simulink model "FW_SkySurfer_HIL"  (R2026b)
settings: Solver=ode4  StopTime=inf  FixedStep=Thil  EnableMultiTasking=on
PreLoadFcn:
  | % Load this folder's HIL settings and MAVLink Bus types (not another project's).
  | run(fullfile(fileparts(get_param(bdroot,'FileName')),'PX4_HIL_preload.m'));
InitFcn:
  | % Record the model first: loading libraries can change the current diagram.
  | assignin('base','lastRunModel',bdroot);
  | % Rebuild HIL settings/Bus types (also after clear all), then aircraft data.
  | hilModelFolder = fileparts(get_param(lastRunModel,'FileName'));
  | run(fullfile(hilModelFolder,'PX4_HIL_preload.m'));
  | run(fullfile(hilModelFolder,'FW_SkySurfer_InitialFunction.m'));
  | clear hilModelFolder
values from neighbouring files (symbols this model uses):
  Aeroelasticity_AIL = [   5   15]    [FW_SkySurfer_InitialFunction.m]
  Aeroelasticity_ELE = [   5   15]    [FW_SkySurfer_InitialFunction.m]
  Aeroelasticity_Gain_AIL = [ 0.8  0.5]    [FW_SkySurfer_InitialFunction.m]
  Aeroelasticity_Gain_ELE = [ 0.9  0.6]    [FW_SkySurfer_InitialFunction.m]
  Aeroelasticity_Gain_RUD = [ 0.9  0.6]    [FW_SkySurfer_InitialFunction.m]
  Aeroelasticity_RUD = [   5   15]    [FW_SkySurfer_InitialFunction.m]
  alpha_avl = [-10 -5 0 5 10 15]    [import_aerostates_avl.m]
  AoA = [-10 -5 0 5 10 15]    [import_aerostates_vsp.m]
  AoS = [-10 0 10]    [import_aerostates_vsp.m]
  b = 1.41    [FW_SkySurfer_InitialFunction.m]
  beta_avl = [-10 -5 0 5 10]    [import_aerostates_avl.m]
  C_wgrp = struct()    [import_aerostates_vsp.m]
  cbar = 0.20    (= 0.2)    [FW_SkySurfer_InitialFunction.m]
  CD_fix_AVL = 0.075    [FW_SkySurfer_InitialFunction.m]
  CD_fix_VSP = 0.065    [FW_SkySurfer_InitialFunction.m]
  CDd01 = zeros(length(mach_avl), length(alpha_avl), length(beta_avl))    [import_aerostates_avl.m]
  CDd02 = zeros(length(mach_avl), length(alpha_avl), length(beta_avl))    [import_aerostates_avl.m]
  CDd03 = zeros(length(mach_avl), length(alpha_avl), length(beta_avl))    [import_aerostates_avl.m]
  CDd04 = zeros(length(mach_avl), length(alpha_avl), length(beta_avl))    [import_aerostates_avl.m]
  CDp = zeros(length(mach_avl), length(alpha_avl), length(beta_avl))    [import_aerostates_avl.m]
  CDq = zeros(length(mach_avl), length(alpha_avl), length(beta_avl))    [import_aerostates_avl.m]
  CDr = zeros(length(mach_avl), length(alpha_avl), length(beta_avl))    [import_aerostates_avl.m]
  CDtot = zeros(length(mach_avl), length(alpha_avl), length(beta_avl))    [import_aerostates_avl.m]
  CG_m = [0.330, 0, 0]    [FW_SkySurfer_InitialFunction.m]
  CLd01 = zeros(length(mach_avl), length(alpha_avl), length(beta_avl))    [import_aerostates_avl.m]
  Cld01 = zeros(length(mach_avl), length(alpha_avl), length(beta_avl))    [import_aerostates_avl.m]
  CLd02 = zeros(length(mach_avl), length(alpha_avl), length(beta_avl))    [import_aerostates_avl.m]
  Cld02 = zeros(length(mach_avl), length(alpha_avl), length(beta_avl))    [import_aerostates_avl.m]
  CLd03 = zeros(length(mach_avl), length(alpha_avl), length(beta_avl))    [import_aerostates_avl.m]
  Cld03 = zeros(length(mach_avl), length(alpha_avl), length(beta_avl))    [import_aerostates_avl.m]
  CLd04 = zeros(length(mach_avl), length(alpha_avl), length(beta_avl))    [import_aerostates_avl.m]
  Cld04 = zeros(length(mach_avl), length(alpha_avl), length(beta_avl))    [import_aerostates_avl.m]
  CLp = zeros(length(mach_avl), length(alpha_avl), length(beta_avl))    [import_aerostates_avl.m]
  Clp = zeros(length(mach_avl), length(alpha_avl), length(beta_avl))    [import_aerostates_avl.m]
  CLq = zeros(length(mach_avl), length(alpha_avl), length(beta_avl))    [import_aerostates_avl.m]
  Clq = zeros(length(mach_avl), length(alpha_avl), length(beta_avl))    [import_aerostates_avl.m]
  CLr = zeros(length(mach_avl), length(alpha_avl), length(beta_avl))    [import_aerostates_avl.m]
  Clr = zeros(length(mach_avl), length(alpha_avl), length(beta_avl))    [import_aerostates_avl.m]
  CLtot = zeros(length(mach_avl), length(alpha_avl), length(beta_avl))    [import_aerostates_avl.m]
  Cltot = zeros(length(mach_avl), length(alpha_avl), length(beta_avl))    [import_aerostates_avl.m]
  Cmd01 = zeros(length(mach_avl), length(alpha_avl), length(beta_avl))    [import_aerostates_avl.m]
  Cmd02 = zeros(length(mach_avl), length(alpha_avl), length(beta_avl))    [import_aerostates_avl.m]
  Cmd03 = zeros(length(mach_avl), length(alpha_avl), length(beta_avl))    [import_aerostates_avl.m]
  Cmd04 = zeros(length(mach_avl), length(alpha_avl), length(beta_avl))    [import_aerostates_avl.m]
  Cmp = zeros(length(mach_avl), length(alpha_avl), length(beta_avl))    [import_aerostates_avl.m]
  Cmq = zeros(length(mach_avl), length(alpha_avl), length(beta_avl))    [import_aerostates_avl.m]
  Cmr = zeros(length(mach_avl), length(alpha_avl), length(beta_avl))    [import_aerostates_avl.m]
  Cmtot = zeros(length(mach_avl), length(alpha_avl), length(beta_avl))    [import_aerostates_avl.m]
  Cnd01 = zeros(length(mach_avl), length(alpha_avl), length(beta_avl))    [import_aerostates_avl.m]
  Cnd02 = zeros(length(mach_avl), length(alpha_avl), length(beta_avl))    [import_aerostates_avl.m]
  Cnd03 = zeros(length(mach_avl), length(alpha_avl), length(beta_avl))    [import_aerostates_avl.m]
  Cnd04 = zeros(length(mach_avl), length(alpha_avl), length(beta_avl))    [import_aerostates_avl.m]
  Cnp = zeros(length(mach_avl), length(alpha_avl), length(beta_avl))    [import_aerostates_avl.m]
  Cnq = zeros(length(mach_avl), length(alpha_avl), length(beta_avl))    [import_aerostates_avl.m]
  Cnr = zeros(length(mach_avl), length(alpha_avl), length(beta_avl))    [import_aerostates_avl.m]
  Cntot = zeros(length(mach_avl), length(alpha_avl), length(beta_avl))    [import_aerostates_avl.m]
  CYd01 = zeros(length(mach_avl), length(alpha_avl), length(beta_avl))    [import_aerostates_avl.m]
  CYd02 = zeros(length(mach_avl), length(alpha_avl), length(beta_avl))    [import_aerostates_avl.m]
  CYd03 = zeros(length(mach_avl), length(alpha_avl), length(beta_avl))    [import_aerostates_avl.m]
  CYd04 = zeros(length(mach_avl), length(alpha_avl), length(beta_avl))    [import_aerostates_avl.m]
  CYp = zeros(length(mach_avl), length(alpha_avl), length(beta_avl))    [import_aerostates_avl.m]
  CYq = zeros(length(mach_avl), length(alpha_avl), length(beta_avl))    [import_aerostates_avl.m]
  CYr = zeros(length(mach_avl), length(alpha_avl), length(beta_avl))    [import_aerostates_avl.m]
  CYtot = zeros(length(mach_avl), length(alpha_avl), length(beta_avl))    [import_aerostates_avl.m]
  del_z = 0    [FW_SkySurfer_InitialFunction.m]
  g = 9.80665    [FW_SkySurfer_InitialFunction.m]
  H0 = 1000 * convlength(1, 'ft', 'm')    [FW_SkySurfer_InitialFunction.m]
  Inertia0 = [  Ixx -Ixy -Ixz  ;                              -Ixy  Iyy -Iyz  ;                              -Ixz -Iyz  Izz ]    [FW_SkySurfer_InitialFunction.m]
  Lat0 = 22.910275834988674    (= 22.910275835)    [FW_SkySurfer_InitialFunction.m]
  Lon0 = 120.31096929726908    (= 120.310969297)    [FW_SkySurfer_InitialFunction.m]
  Mach = [0.05 0.10]    [import_aerostates_vsp.m]
  mach_avl = [0.05 0.10]    [import_aerostates_avl.m]
  Mass0 = 1.3    [FW_SkySurfer_InitialFunction.m]
  Phi0 = 0    [FW_SkySurfer_InitialFunction.m]
  Psi0 = 0    [FW_SkySurfer_InitialFunction.m]
  Psi_w = 0    [FW_SkySurfer_InitialFunction.m]
  Theta0 = 0.8633    [FW_SkySurfer_InitialFunction.m]
  Thil = 1/250    (= 0.004)    [FW_SkySurfer_InitialFunction.m]
  U0 = 40.0309 * convvel(1, 'kts', 'm/s')    [FW_SkySurfer_InitialFunction.m]
  useAVL_VSP = 0    [FW_SkySurfer_InitialFunction.m]
  V0 = 0    [FW_SkySurfer_InitialFunction.m]
  Vel_w = 0    [FW_SkySurfer_InitialFunction.m]
  W0 = 0.6032 * convvel(1, 'kts', 'm/s')    [FW_SkySurfer_InitialFunction.m]
  XREF_m = [0.330, 0, 0]    [FW_SkySurfer_InitialFunction.m]
undefined symbols (not defined in the file or in its folder): F, Light, m, MIL, Newton, Raphson, s, Ts, uavData
libraries: simulink_extras x28, aerolibasang x5, shared6dofsys x4, aerolibwind2 x4, sharedtransform x3, sharedutil x2, shared6dof x2, simulink x1, aerolibatmos2 x1, aerolibconvert2 x1
(part 1 of 3)
settings Model: Creator=master  LastModifiedBy=iec
settings SolverCC: AutoInsertRateTranBlk=on
settings DataIOCC: DSMLogging=off  ReturnWorkspaceOutputs=off  SaveFormat=Structure  SaveOutput=off  SaveTime=off  SignalLogging=off  SignalLoggingSaveFormat=ModelDataLogs
settings OptimizationCC: DefaultParameterBehavior=Inlined  DifferentSizesBufferReuse=on  EnhancedBackFolding=on  OptimizationCustomize=off  OptimizeBlockOrder=speed  SimCompilerOptimization=on
settings DebuggingCC: ArithmeticOperatorsInVariantConditions=warning  FcnCallInpInsideContextMsg=warning  MergeDetectMultiDrivingBlocksExec=none  MultiTaskCondExecSysMsg=none  ParameterTunabilityLossMsg=error  SFExecutionAtInitializationDiag=none  SFNoUnconditionalDefaultTransitionDiag=warning  SFUnexpectedBacktrackingDiag=warning
settings HardwareCC: ProdHWDeviceType=Apple->ARM64  ProdLongLongMode=on
settings SFSimCC: CustomCodeUndefinedFunction=UseInterfaceOnly  MATLABDynamicMemAlloc=off  SimAnalyzeCustomCode=on  SimUseLocalCustomCode=off
settings RTWCC: DLArmComputeVersion=19.05  GenerateReport=on  LaunchReport=on  RTWUseLocalCustomCode=off
settings CodeAppCC: ForceParamTrailComments=on  OperatorAnnotations=on
settings GRTTargetCC: TargetLangStandard=C89/C90 (ANSI)
settings ConfigComp: CovExternalEMLEnable=off  CovSaveCumulativeToWorkspaceVar=on  CovSaveSingleToWorkspaceVar=on
settings SimscapeCC: SimscapeNormalizeSystem=off  SimscapeUseEnergyAccounting=off

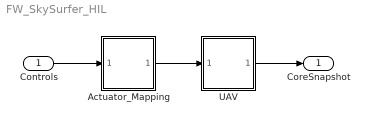
== system FW_SkySurfer_HIL ==
  Controls : Inport  PortDimensions=16  SampleTime=Thil  Interpolate=off
  Actuator_Mapping : Subsystem
  UAV : Subsystem
  CoreSnapshot : Outport
  wires:
  Actuator_Mapping/1(CS_OUT) -> UAV/1(CS_OUT)
  Controls/1 -> Actuator_Mapping/1(ActuatorControls)
  UAV/1(CoreSnapshot) -> CoreSnapshot/1

== system FW_SkySurfer_HIL/Actuator_Mapping ==
  ActuatorControls : Inport
  Constant : Constant
  Demux : Demux  Outputs=5
  Select_Channels : Selector  InputPortWidth=16  IndexOptions=Index vector (dialog)  Indices=[1 2 3 4 5]  OutputSizes=1
  Bus Element Out : Outport  PortName=CS_OUT  Element=ARM
  Bus Element Out1 : Outport  PortName=CS_OUT  Element=FW_THR
  Bus Element Out2 : Outport  PortName=CS_OUT  Element=FW_AIL_R
  Bus Element Out3 : Outport  PortName=CS_OUT  Element=FW_AIL_L
  Bus Element Out4 : Outport  PortName=CS_OUT  Element=FW_ELE
  Bus Element Out5 : Outport  PortName=CS_OUT  Element=FW_RUD
  wires:
  Constant/1 -> Bus Element Out/1
  ActuatorControls/1 -> Select_Channels/1
  Select_Channels/1 -> Demux/1
  Demux/1 -> Bus Element Out3/1
  Demux/2 -> Bus Element Out2/1
  Demux/3 -> Bus Element Out4/1
  Demux/4 -> Bus Element Out5/1
  Demux/5 -> Bus Element Out1/1

== system FW_SkySurfer_HIL/UAV ==
  CS_OUT : Inport
  ACTUATOR : Subsystem
  SETTING1 : Subsystem  DataTypeOverride=Double  DataTypeOverrideAppliesTo=Floating-point
  UAV : Subsystem  SystemSampleTime=Ts
      settings: RTWFcnNameOpts=Use subsystem name
  CoreSnapshot : Outport
  wires:
  UAV/1(CoreSnapshot) -> CoreSnapshot/1
  SETTING1/2(SIM_SET) -> UAV/2(SIM_SET)  "SIM_SET_"
  SETTING1/1(INI_COND) -> UAV/1(INI_COND)  "INI_COND_"
  ACTUATOR/1(Actuator) -> UAV/3(Actuator)
  CS_OUT/1 -> ACTUATOR/1(CS_OUT)  "CS_OUT"

== system FW_SkySurfer_HIL/UAV/ACTUATOR ==
  Bus Element In1 : Inport  PortName=CS_OUT  Element=FW_AIL_R
  Bus Element In2 : Inport  PortName=CS_OUT  Element=FW_AIL_L
  Bus Element In3 : Inport  PortName=CS_OUT  Element=FW_ELE
  Bus Element In4 : Inport  PortName=CS_OUT  Element=FW_THR
  Bus Element In5 : Inport  PortName=CS_OUT  Element=FW_RUD
  Gain : Gain  Gain=27
  Gain1 : Gain  Gain=35
  Gain2 : Gain  Gain=30
  Gain3 : Gain  Gain=-1
  Gain4 : Gain  Gain=-1
  Gain5 : Gain
  Gain6 : Gain  Gain=30
  Gain8 : Gain
  Limit_AIL_L : Saturate  UpperLimit=1  LowerLimit=-1
  Limit_AIL_R : Saturate  UpperLimit=1  LowerLimit=-1
  Limit_ELE : Saturate  UpperLimit=1  LowerLimit=-1
  Limit_RUD : Saturate  UpperLimit=1  LowerLimit=-1
  Limit_THR : Saturate  UpperLimit=1  LowerLimit=0
  Rate Limiter{,1..3} (4 alike) : RateLimiter  RisingSlewLimit=500  FallingSlewLimit=-500  SampleTimeMode=inherited
  Transfer Fcn{,1..2,4} (4 alike) : TransferFcn  Numerator=[20]  Denominator=[1 20]
  Transfer Fcn3 : TransferFcn  Numerator=[5]  Denominator=[1 5]
  Out Bus Element : Outport  PortName=Actuator  Element=Aileron_R
  Out Bus Element1 : Outport  PortName=Actuator  Element=Aileron_L
  Out Bus Element2 : Outport  PortName=Actuator  Element=Elevator
  Out Bus Element3 : Outport  PortName=Actuator  Element=Throttle
  Out Bus Element4 : Outport  PortName=Actuator  Element=Rudder
  wires:
  Transfer Fcn/1 -> Rate Limiter/1  "Ail_R"
  Transfer Fcn1/1 -> Rate Limiter1/1  "Ele"
  Transfer Fcn2/1 -> Rate Limiter2/1  "Rud"
  Gain4/1 -> Out Bus Element2/1
  Gain5/1 -> Out Bus Element/1
  Rate Limiter/1 -> Gain5/1
  Rate Limiter1/1 -> Gain4/1
  Rate Limiter2/1 -> Gain8/1
  Rate Limiter3/1 -> Gain3/1
  Transfer Fcn4/1 -> Rate Limiter3/1  "Ail_L"
  Gain3/1 -> Out Bus Element1/1
  Gain8/1 -> Out Bus Element4/1
  Limit_RUD/1 -> Gain1/1
  Bus Element In5/1 -> Limit_RUD/1
  Limit_THR/1 -> Transfer Fcn3/1
  Bus Element In4/1 -> Limit_THR/1
  Limit_ELE/1 -> Gain/1
  Bus Element In3/1 -> Limit_ELE/1
  Limit_AIL_L/1 -> Gain2/1
  Bus Element In2/1 -> Limit_AIL_L/1
  Limit_AIL_R/1 -> Gain6/1
  Bus Element In1/1 -> Limit_AIL_R/1
  Gain2/1 -> Transfer Fcn4/1
  Gain/1 -> Transfer Fcn1/1
  Gain1/1 -> Transfer Fcn2/1
  Gain6/1 -> Transfer Fcn/1
  Transfer Fcn3/1 -> Out Bus Element3/1  "Thr"

== system FW_SkySurfer_HIL/UAV/SETTING1 ==
  Bus Creator : BusCreator  Inputs=12
  Bus Creator1 : BusCreator  Inputs=4
  const1 : Constant  Value=Mass0
  const10 : Constant  Value=Psi0
  const11 : Constant  Value=Lat0
  const12 : Constant  Value=Lon0
  const13 : Constant  Value=H0
  const15 : Constant  Value=Vel_w
  const16 : Constant  Value=Psi_w
  const17 : Constant
  const18 : Constant
  const2 : Constant  Value=Inertia0
  const4 : Constant  Value=CG_m(1)
  const5 : Constant  Value=U0
  const6 : Constant  Value=V0
  const7 : Constant  Value=W0
  const8 : Constant  Value=Phi0
  const9 : Constant  Value=Theta0
  INI_COND : Outport
  SIM_SET : Outport  Port=2
  wires:
  Bus Creator/1 -> INI_COND/1
  const1/1 -> Bus Creator/1  "Mass0"
  const2/1 -> Bus Creator/2  "Inertia0"
  const4/1 -> Bus Creator/3  "CG0"
  const5/1 -> Bus Creator/4  "U0"
  const9/1 -> Bus Creator/8  "Theta0"
  const10/1 -> Bus Creator/9  "Psi0"
  const11/1 -> Bus Creator/10  "Latitude0"
  const12/1 -> Bus Creator/11  "Longitude0"
  const13/1 -> Bus Creator/12  "Alt0"
  Bus Creator1/1 -> SIM_SET/1
  const8/1 -> Bus Creator/7  "Phi0"
  const6/1 -> Bus Creator/5  "V0"
  const7/1 -> Bus Creator/6  "W0"
  const16/1 -> Bus Creator1/2  "PsiWind"
  const17/1 -> Bus Creator1/3  "IdxWind"
  const15/1 -> Bus Creator1/1  "VelWind"
  const18/1 -> Bus Creator1/4  "IdxAirport"

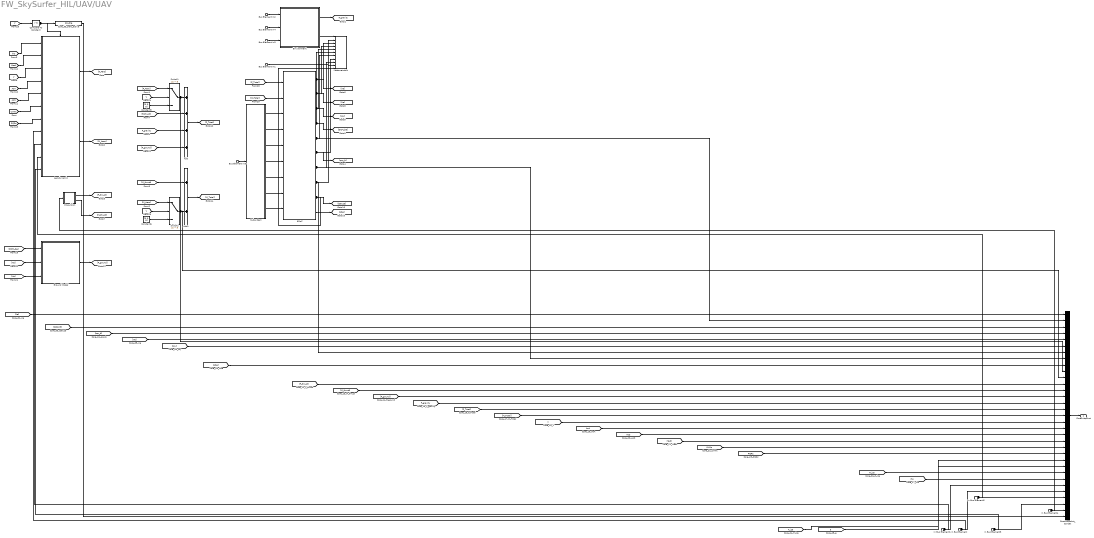
== system FW_SkySurfer_HIL/UAV/UAV ==
  Bus Element In1 : Inport  PortName=INI_COND
  Bus Element In5 : Inport  PortName=INI_COND
  Bus Element In2 : Inport  Port=2  PortName=SIM_SET  Element=IdxWind
  Bus Element In3 : Inport  Port=2  PortName=SIM_SET  Element=PsiWind
  Bus Element In4 : Inport  Port=2  PortName=SIM_SET  Element=VelWind
  In Bus Element : Inport  Port=3  PortName=Actuator  Element=Aileron_R
  In Bus Element1 : Inport  Port=3  PortName=Actuator  Element=Aileron_L
  In Bus Element2 : Inport  Port=3  PortName=Actuator  Element=Elevator
  In Bus Element3 : Inport  Port=3  PortName=Actuator  Element=Rudder
  In Bus Element4 : Inport  Port=3  PortName=Actuator  Element=Throttle
  6DoF : Subsystem
  Add : Sum  Inputs=++++
  Add1 : Sum
  Aerodynamic : Subsystem
  Compare To Constant : simulink/Logic and Bit Operations/Compare To Constant  relop=>  const=5  OutDataTypeStr=boolean
  Constant5 : Constant  Value=[0 0 0]
  Constant6 : Constant  Value=[0 0 0]
  CoreSnapshot_Concat : Concatenate  NumInputs=33
  Core_33_aero_active : DataTypeConversion  OutDataTypeStr=double  SaturateOnIntegerOverflow=off  RndMeth=Floor
  Environment : Subsystem
  Ground Model : Subsystem
  Measurement : Subsystem
  Propulsion : Subsystem
  Subsystem : Subsystem
  Switch1 : Switch  Criteria=u2 > Threshold  Threshold=5  SaturateOnIntegerOverflow=off  InputSameDT=off
  Switch2 : Switch  Criteria=u2 > Threshold  Threshold=5  SaturateOnIntegerOverflow=off  InputSameDT=off
  CoreSnapshot : Outport
  tag scope: F_gravity=global
  wires:
  [F_gravity] -> Add/3
  Aerodynamic/1(F_aero) -> [F_Aero]
  Aerodynamic/2(M_aero) -> [M_Aero]
  [AoA] -> Aerodynamic/4(AoA (deg))
  [AoS] -> Aerodynamic/5(AoS (deg))
  [UVWc] -> Aerodynamic/6(UVW(m/s))
  [PQRc] -> Aerodynamic/7(PQRc (rad/s))
  [M_thrust] -> Add1/1
  [DCM_be] -> Ground Model/1(DCMbe)
  [Xe] -> Ground Model/2(Xe)
  [Ve] -> Ground Model/3(Ve)
  Ground Model/1(Fb_contact) -> [F_gound]
  [rho] -> Aerodynamic/1(rho(kg/m^3))
  [Mach] -> Aerodynamic/2(Mach)
  [V] -> Aerodynamic/3(Vt (m/s))
  [F_gound] -> Add/4
  [F_thrust] -> Add/2
  Add/1 -> [F_Total]
  Add1/1 -> [M_Total]
  Subsystem/5(VB0) -> 6DoF/7(VB0)
  Subsystem/2(mass) -> 6DoF/4(mass)
  Environment/1(F_gravity) -> [F_gravity]
  Bus Element In2/1 -> Environment/1(WIND_IDX)
  [F_Total] -> 6DoF/1(Forces)
  Bus Element In5/1 -> Subsystem/1(INI_COND)
  Subsystem/7(XE0) -> 6DoF/9(XE0)
  Bus Element In4/1 -> Environment/2(wind.Vel)
  Subsystem/1(m_dot) -> 6DoF/3(m_dot)
  Subsystem/4(I) -> 6DoF/6(I)
  [M_Total] -> 6DoF/2(Moments)
  6DoF/10(Abe) -> [Abe]
  Bus Element In3/1 -> Environment/3(wind.Psi)
  Subsystem/3(I_dot) -> 6DoF/5(I_dot)
  Subsystem/6(EA0) -> 6DoF/8(EA0)
  [V] -> Compare To Constant/1
  Propulsion/1(F_thr) -> [F_thrust]
  Propulsion/2(M_thr) -> [M_thrust]
  In Bus Element4/1 -> Propulsion/1(Throttle (0-1)), CoreSnapshot_Concat/32
  In Bus Element/1 -> Aerodynamic/8(Aileron_R (deg)), CoreSnapshot_Concat/29
  In Bus Element3/1 -> Aerodynamic/11(Rudder (deg)), CoreSnapshot_Concat/31
  In Bus Element2/1 -> Aerodynamic/10(Elevator (deg)), CoreSnapshot_Concat/30
  In Bus Element1/1 -> Aerodynamic/9(Aileron_L (deg)), CoreSnapshot_Concat/28
  [V] -> Switch1/2
  [F_Aero] -> Switch1/1
  Constant5/1 -> Switch1/3
  Switch1/1 -> Add/1, CoreSnapshot_Concat/10
  Constant6/1 -> Switch2/3
  [V] -> Switch2/2
  [M_Aero] -> Switch2/1
  Switch2/1 -> Add1/2, CoreSnapshot_Concat/11
  6DoF/2(Xe) -> [Xe], Measurement/4(XE)
  6DoF/6(p,q,r) -> [pqr_b], Measurement/8(AR)
  6DoF/7(Ab) -> Measurement/9(AB), CoreSnapshot_Concat/8
  6DoF/5(Vb) -> Measurement/7(VB), CoreSnapshot_Concat/2
  6DoF/8(pdot,qdot,rdot) -> Measurement/10(AA), CoreSnapshot_Concat/7
  6DoF/4(DCM) -> [DCM_be], Measurement/6(DCM)
  Bus Element In1/1 -> Measurement/2(INI_COND)
  Environment/2(WIND) -> Measurement/1(WIND)
  6DoF/3(Euler) -> [rpy], Measurement/5(EA)
  6DoF/1(Ve) -> [Ve], Measurement/3(VE)
  6DoF/9(Q0123) -> [Q0123], Measurement/11(Q0123)
  Compare To Constant/1 -> Aerodynamic/Enable, Core_33_aero_active/1
  CoreSnapshot_Concat/1 -> CoreSnapshot/1
  [Xe] -> CoreSnapshot_Concat/1
  [Q0123] -> CoreSnapshot_Concat/3
  [pqr_b] -> CoreSnapshot_Concat/4
  [Ve] -> CoreSnapshot_Concat/5
  [rpy] -> CoreSnapshot_Concat/6
  [Abe] -> CoreSnapshot_Concat/9
  [F_thrust] -> CoreSnapshot_Concat/12
  [M_thrust] -> CoreSnapshot_Concat/13
  [F_gound] -> CoreSnapshot_Concat/14
  [F_gravity] -> CoreSnapshot_Concat/15
  [F_Total] -> CoreSnapshot_Concat/16
  [M_Total] -> CoreSnapshot_Concat/17
  [V] -> CoreSnapshot_Concat/18
  [AoA] -> CoreSnapshot_Concat/19
  [AoS] -> CoreSnapshot_Concat/20
  [Mach] -> CoreSnapshot_Concat/21
  [UVWc] -> CoreSnapshot_Concat/22
  [PQRc] -> CoreSnapshot_Concat/23
  [T_isa] -> CoreSnapshot_Concat/24
  [a] -> CoreSnapshot_Concat/25
  [P_isa] -> CoreSnapshot_Concat/26
  [rho] -> CoreSnapshot_Concat/27
  Core_33_aero_active/1 -> CoreSnapshot_Concat/33

== system FW_SkySurfer_HIL/UAV/UAV/6DoF ==
  Forces : Inport  Unit=lb  PortDimensions=3
  Moments : Inport  Port=2  Unit=lb*ft  PortDimensions=3
  m_dot : Inport  Port=3  Unit=slug/s  PortDimensions=1
  mass : Inport  Port=4  Unit=slug  PortDimensions=1
  I_dot : Inport  Port=5  Unit=slug*ft^2/s  PortDimensions=[3 3]
  I : Inport  Port=6  Unit=slug*ft^2  PortDimensions=[3 3]
  VB0 : Inport  Port=7  PortDimensions=3
  EA0 : Inport  Port=8  PortDimensions=3
  XE0 : Inport  Port=9  PortDimensions=3
  Ground : Ground  Commented=on
  PQR : Integrator
  Product : Product  Inputs=*/  OutDataTypeStr=double  SaturateOnIntegerOverflow=on
  Subsystem : Subsystem
  Subsystem1 : Subsystem
  Subsystem2 : Subsystem
  Sum : Sum  Inputs=|++  SaturateOnIntegerOverflow=on
  Terminator : Terminator
  Transpose : Math  Operator=transpose  SignedPower=on
  UVWb : Integrator  InitialConditionSource=external
  Vbxw : sharedutil/3x3 Cross Product  aMode=aMode
  Velocity Conversion2 : shared6dof/6DOF (Euler Angles)/Velocity Conversion2  Commented=on  SystemSampleTime=-1  VariantActivationTime=update diagram  EmptyChoice=off  PassThrough=off  PassThroughVariantControl=(default)  EmptyChoiceVariantControl=(default)  AllowFlexibleInterface=on  Latency=0  AutoFrameSizeCalculation=off
  XYZe : Integrator  InitialConditionSource=external
  "transform to Inertial axes " : shared6dof/6DOF (Euler Angles)/transform to Inertial axes   SystemSampleTime=-1  VariantActivationTime=update diagram  EmptyChoice=off  PassThrough=off  PassThroughVariantControl=(default)  EmptyChoiceVariantControl=(default)  AllowFlexibleInterface=on  Latency=0  AutoFrameSizeCalculation=off
  Ve : Outport  PortDimensions=3  VectorParamsAs1DForOutWhenUnconnected=off
  Xe : Outport  Port=2  PortDimensions=3  VectorParamsAs1DForOutWhenUnconnected=off
  Euler : Outport  Port=3  Unit=rad  PortDimensions=3  VectorParamsAs1DForOutWhenUnconnected=off
  DCM : Outport  Port=4  Unit=1  PortDimensions=[3 3]  VectorParamsAs1DForOutWhenUnconnected=off
  Vb : Outport  Port=5  Unit=ft/s  PortDimensions=3  VectorParamsAs1DForOutWhenUnconnected=off
  p,q,r : Outport  Port=6  Unit=rad/s  PortDimensions=3  VectorParamsAs1DForOutWhenUnconnected=off
  Ab : Outport  Port=7  Unit=ft/s^2  PortDimensions=3  VectorParamsAs1DForOutWhenUnconnected=off
  pdot,qdot,rdot : Outport  Port=8  Unit=rad/s^2  PortDimensions=3  VectorParamsAs1DForOutWhenUnconnected=off
  Q0123 : Outport  Port=9  VectorParamsAs1DForOutWhenUnconnected=off
  Abe : Outport  Port=10  Unit=ft/s^2  PortDimensions=3  VectorParamsAs1DForOutWhenUnconnected=off
  wires:
  Subsystem/1(DCM) -> Transpose/1, DCM/1
  EA0/1 -> Subsystem/2(eul_0)
  mass/1 -> Subsystem1/3("mass ")
  Subsystem/2(Euler) -> Euler/1
  m_dot/1 -> Subsystem1/4(mdot)
  Ground/1 -> Velocity Conversion2/1
  I/1 -> Subsystem1/5(I)
  Transpose/1 -> "transform to Inertial axes "/2
  Velocity Conversion2/1 -> Subsystem1/1(Vre)
  Subsystem1/3("I, I_dot ") -> Subsystem2/2("I, I_dot")
  I_dot/1 -> Subsystem1/6(I_dot)
  Vbxw/1 -> Sum/2
  "transform to Inertial axes "/1 -> Ve/1, XYZe/1
  Subsystem1/1("forces ") -> Product/1
  Subsystem1/2(mass) -> Product/2
  Subsystem1/4(Out1) -> Terminator/1
  Moments/1 -> Subsystem2/3(Moments)
  Forces/1 -> Subsystem1/2(forces)
  Subsystem2/1(pdot qdot rdot) -> pdot,qdot,rdot/1, PQR/1
  Sum/1 -> Ab/1, UVWb/1
  Subsystem/3(Q) -> Q0123/1
  Product/1 -> Abe/1, Sum/1
  PQR/1 -> Subsystem2/1(p q r), p,q,r/1, Vbxw/2, Subsystem/1(p q r)
  VB0/1 -> UVWb/2
  UVWb/1 -> Vb/1, "transform to Inertial axes "/1, Vbxw/1
  XE0/1 -> XYZe/2
  XYZe/1 -> Xe/1

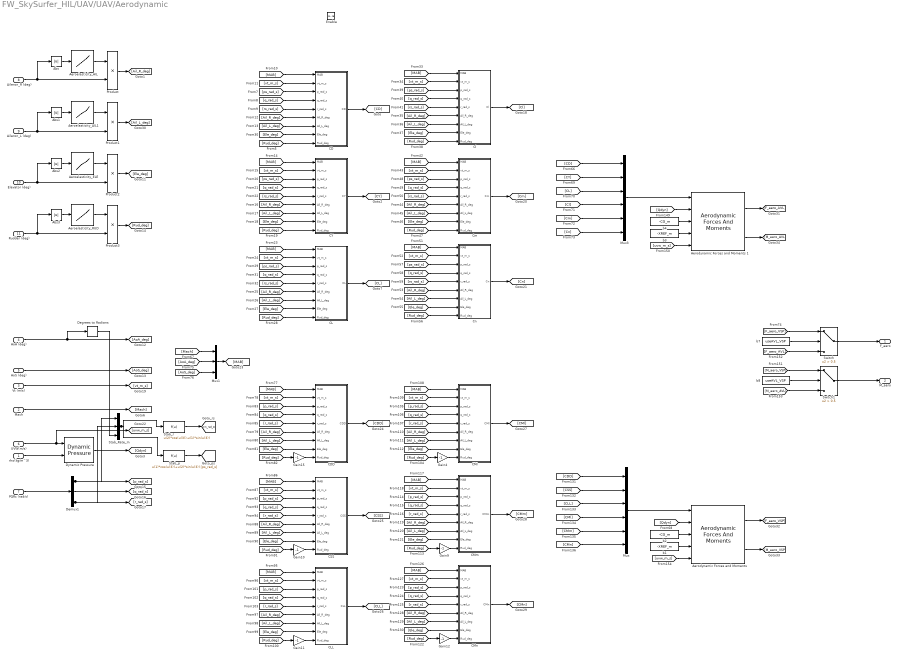
== system FW_SkySurfer_HIL/UAV/UAV/Aerodynamic ==
  rho(kg/m^3) : Inport
  Mach : Inport  Port=2
  Vt (m/s) : Inport  Port=3
  AoA (deg) : Inport  Port=4
  AoS (deg) : Inport  Port=5
  UVW(m/s) : Inport  Port=6
  PQRc (rad/s) : Inport  Port=7
  Aileron_R (deg) : Inport  Port=8
  Aileron_L (deg) : Inport  Port=9
  Elevator (deg) : Inport  Port=10
  Rudder (deg) : Inport  Port=11
  Enable : EnablePort
  Abs{,1..3} (4 alike) : Abs  SaturateOnIntegerOverflow=off
  "Aerodynamic Forces and Moments " : AerodynamicForcesAndMoments  inputAxes=Wind  S=S  b=b  cbar=cbar
  Aerodynamic Forces and Moments 1 : AerodynamicForcesAndMoments  inputAxes=Stability  S=S  b=b  cbar=cbar
  Aeroelasticity_AIL : Lookup_n-D  NumberOfTableDimensions=1  BreakpointsForDimension1=Aeroelasticity_AIL  BreakpointsForDimension3=[5, 7]  Table=Aeroelasticity_Gain_AIL  ExtrapMethod=Clip  InternalRulePriority=Speed  RndMeth=Simplest
  Aeroelasticity_AIL1 : Lookup_n-D  NumberOfTableDimensions=1  BreakpointsForDimension1=Aeroelasticity_AIL  BreakpointsForDimension3=[5, 7]  Table=Aeroelasticity_Gain_AIL  ExtrapMethod=Clip  InternalRulePriority=Speed  RndMeth=Simplest
  Aeroelasticity_ELE : Lookup_n-D  NumberOfTableDimensions=1  BreakpointsForDimension1=Aeroelasticity_ELE  BreakpointsForDimension3=[5, 7]  Table=Aeroelasticity_Gain_ELE  ExtrapMethod=Clip  InternalRulePriority=Speed  RndMeth=Simplest
  Aeroelasticity_RUD : Lookup_n-D  NumberOfTableDimensions=1  BreakpointsForDimension1=Aeroelasticity_RUD  BreakpointsForDimension3=[5, 7]  Table=Aeroelasticity_Gain_RUD  ExtrapMethod=Clip  InternalRulePriority=Speed  RndMeth=Simplest
  CD : Subsystem
  CDD : Subsystem
  CL : Subsystem
  CLL : Subsystem
  CMl : Subsystem
  CMm : Subsystem
  CMn : Subsystem
  CSS : Subsystem
  CY : Subsystem
  Cl : Subsystem
  Cm : Subsystem
  Cn : Subsystem
  Degrees to Radians : simulink_extras/Transformations/Degrees to Radians
  Demux1 : Demux  Outputs=3
  Dynamic Pressure : aerolibasang/Dynamic Pressure
  Gain{4,9..12,15} (6 alike) : Gain  Gain=-1
  Mux : Mux  Inputs=6
  Mux1 : Mux  Inputs=3
  Mux3 : Mux  Inputs=6
  Product{,1..3} (4 alike) : Product
  Stab_Rate_In : Mux  Inputs=3
  Stab_p : Fcn  Expr=u(1)*cos(u(3))+u(2)*sin(u(3))
  Stab_r : Fcn  Expr=u(2)*cos(u(3))-u(1)*sin(u(3))
  Switch : Switch  Criteria=u2 > Threshold  Threshold=0.5  SaturateOnIntegerOverflow=off  InputSameDT=off
  Switch1 : Switch  Criteria=u2 > Threshold  Threshold=0.5  SaturateOnIntegerOverflow=off  InputSameDT=off
  b1 : Constant  Value=-XREF_m
  b2 : Constant  Value=-CG_m
  b3 : Constant  Value=-XREF_m
  b4 : Constant  Value=-CG_m
  b7 : Constant  Value=useAVL_VSP
  b8 : Constant  Value=useAVL_VSP
  F_aero : Outport  Unit=N
  M_aero : Outport  Port=2
  wires:
  Demux1/2 -> [q_rad_s]
  rho(kg/m^3)/1 -> Dynamic Pressure/2
  Vt (m/s)/1 -> [vt_m_s]
  PQRc (rad/s)/1 -> Demux1/1
  UVW(m/s)/1 -> Dynamic Pressure/1, [uvw_m_s]
  Dynamic Pressure/1 -> [Qdyn]
  AoA (deg)/1 -> [AoA_deg], Degrees to Radians/1
  AoS (deg)/1 -> [AoS_deg]
  Mach/1 -> [Mach]
  CD/1(CD) -> [CD]
  CY/1(CY) -> [CY]
  CL/1(CL) -> [CL]
  Cl/1(Cl) -> [Cl]
  Cm/1(Cm) -> [Cm]
  Cn/1(Cn) -> [Cn]
  [CMm] -> Mux/5
  [CMn] -> Mux/6
  b1/1 -> "Aerodynamic Forces and Moments "/4
  [CMl] -> Mux/4
  [Qdyn] -> "Aerodynamic Forces and Moments "/2
  b2/1 -> "Aerodynamic Forces and Moments "/3
  [AoA_deg] -> Mux1/2
  [Mach] -> Mux1/1
  [AoS_deg] -> Mux1/3
  Mux1/1 -> [MAB]
  CDD/1(CDD) -> [CDD]
  [MAB] -> CDD/1(MAB)
  [vt_m_s] -> CDD/2(vt_m_s)
  [p_rad_s] -> CDD/3(p_rad_s)
  [q_rad_s] -> CDD/4(q_rad_s)
  [r_rad_s] -> CDD/5(r_rad_s)
  [Ail_R_deg] -> CDD/6(Ail_R_deg)
  [Ail_L_deg] -> CDD/7(Ail_L_deg)
  [Ele_deg] -> CDD/8(Ele_deg)
  [Rud_deg] -> Gain15/1
  [MAB] -> CSS/1(MAB)
  [vt_m_s] -> CSS/2(vt_m_s)
  [p_rad_s] -> CSS/3(p_rad_s)
  [q_rad_s] -> CSS/4(q_rad_s)
  [r_rad_s] -> CSS/5(r_rad_s)
  [Ail_R_deg] -> CSS/6(Ail_R_deg)
  [Ail_L_deg] -> CSS/7(Ail_L_deg)
  [Ele_deg] -> CSS/8(Ele_deg)
  [Rud_deg] -> Gain10/1
  [MAB] -> CLL/1(MAB)
  [vt_m_s] -> CLL/2(vt_m_s)
  [p_rad_s] -> CLL/3(p_rad_s)
  [q_rad_s] -> CLL/4(q_rad_s)
  [r_rad_s] -> CLL/5(r_rad_s)
  [Ail_R_deg] -> CLL/6(Ail_R_deg)
  [Ail_L_deg] -> CLL/7(Ail_L_deg)
  [Ele_deg] -> CLL/8(Ele_deg)
  [Rud_deg] -> Gain11/1
  CSS/1(CSS) -> [CSS]
  CLL/1(CLL) -> [CLL]
  CMl/1(CMl) -> [CMl]
  CMm/1(CMm) -> [CMm]
  CMn/1(CMn) -> [CMn]
  [MAB] -> CMl/1(MAB)
  [vt_m_s] -> CMl/2(vt_m_s)
  [p_rad_s] -> CMl/3(p_rad_s)
  [q_rad_s] -> CMl/4(q_rad_s)
  [r_rad_s] -> CMl/5(r_rad_s)
  [Ail_R_deg] -> CMl/6(Ail_R_deg)
  [Ail_L_deg] -> CMl/7(Ail_L_deg)
  [Ele_deg] -> CMl/8(Ele_deg)
  [Rud_deg] -> Gain4/1
  [MAB] -> CMm/1(MAB)
  [vt_m_s] -> CMm/2(vt_m_s)
  [p_rad_s] -> CMm/3(p_rad_s)
  [q_rad_s] -> CMm/4(q_rad_s)
  [r_rad_s] -> CMm/5(r_rad_s)
  [Ail_R_deg] -> CMm/6(Ail_R_deg)
  [Ail_L_deg] -> CMm/7(Ail_L_deg)
  [Ele_deg] -> CMm/8(Ele_deg)
  [Rud_deg] -> Gain9/1
  [MAB] -> CMn/1(MAB)
  [vt_m_s] -> CMn/2(vt_m_s)
  [p_rad_s] -> CMn/3(p_rad_s)
  [q_rad_s] -> CMn/4(q_rad_s)
  [r_rad_s] -> CMn/5(r_rad_s)
  [Ail_R_deg] -> CMn/6(Ail_R_deg)
  [Ail_L_deg] -> CMn/7(Ail_L_deg)
  [Ele_deg] -> CMn/8(Ele_deg)
  [Rud_deg] -> Gain12/1
  [Ele_deg] -> CD/8(Ele_deg)
  [Ail_L_deg] -> CD/7(Ail_L_deg)
  [Ail_R_deg] -> CD/6(Ail_R_deg)
  [rs_rad_s] -> CD/5(r_rad_s)
  [q_rad_s] -> CD/4(q_rad_s)
  [ps_rad_s] -> CD/3(p_rad_s)
  [vt_m_s] -> CD/2(vt_m_s)
  [MAB] -> CD/1(MAB)
  [MAB] -> CY/1(MAB)
  [vt_m_s] -> CY/2(vt_m_s)
  [ps_rad_s] -> CY/3(p_rad_s)
  [q_rad_s] -> CY/4(q_rad_s)
  [rs_rad_s] -> CY/5(r_rad_s)
  [Ail_R_deg] -> CY/6(Ail_R_deg)
  [Ail_L_deg] -> CY/7(Ail_L_deg)
  [Ele_deg] -> CY/8(Ele_deg)
  [MAB] -> CL/1(MAB)
  [vt_m_s] -> CL/2(vt_m_s)
  [ps_rad_s] -> CL/3(p_rad_s)
  [q_rad_s] -> CL/4(q_rad_s)
  [rs_rad_s] -> CL/5(r_rad_s)
  [Ail_R_deg] -> CL/6(Ail_R_deg)
  [Ail_L_deg] -> CL/7(Ail_L_deg)
  [Ele_deg] -> CL/8(Ele_deg)
  [MAB] -> Cl/1(MAB)
  [vt_m_s] -> Cl/2(vt_m_s)
  [ps_rad_s] -> Cl/3(p_rad_s)
  [q_rad_s] -> Cl/4(q_rad_s)
  [rs_rad_s] -> Cl/5(r_rad_s)
  [Ail_R_deg] -> Cl/6(Ail_R_deg)
  [Ail_L_deg] -> Cl/7(Ail_L_deg)
  [Ele_deg] -> Cl/8(Ele_deg)
  [MAB] -> Cm/1(MAB)
  [vt_m_s] -> Cm/2(vt_m_s)
  [ps_rad_s] -> Cm/3(p_rad_s)
  [q_rad_s] -> Cm/4(q_rad_s)
  [rs_rad_s] -> Cm/5(r_rad_s)
  [Ail_R_deg] -> Cm/6(Ail_R_deg)
  [Ail_L_deg] -> Cm/7(Ail_L_deg)
  [Ele_deg] -> Cm/8(Ele_deg)
  [MAB] -> Cn/1(MAB)
  [vt_m_s] -> Cn/2(vt_m_s)
  [ps_rad_s] -> Cn/3(p_rad_s)
  [q_rad_s] -> Cn/4(q_rad_s)
  [rs_rad_s] -> Cn/5(r_rad_s)
  [Ail_R_deg] -> Cn/6(Ail_R_deg)
  [Ail_L_deg] -> Cn/7(Ail_L_deg)
  [Ele_deg] -> Cn/8(Ele_deg)
  [Cl] -> Mux3/4
  [CD] -> Mux3/1
  [Cn] -> Mux3/6
  [Cm] -> Mux3/5
  [CL] -> Mux3/3
  [Rud_deg] -> CD/9(Rud_deg)
  [Rud_deg] -> CY/9(Rud_deg)
  [Rud_deg] -> CL/9(Rud_deg)
  [Rud_deg] -> Cn/9(Rud_deg)
  [Rud_deg] -> Cm/9(Rud_deg)
  [Rud_deg] -> Cl/9(Rud_deg)
  b4/1 -> Aerodynamic Forces and Moments 1/3
  [Qdyn] -> Aerodynamic Forces and Moments 1/2
  b3/1 -> Aerodynamic Forces and Moments 1/4
  [uvw_m_s] -> Aerodynamic Forces and Moments 1/5
  [CDD] -> Mux/1
  [CLL] -> Mux/3
  Mux3/1 -> Aerodynamic Forces and Moments 1/1
  [CSS] -> Mux/2
  Mux/1 -> "Aerodynamic Forces and Moments "/1
  "Aerodynamic Forces and Moments "/1 -> [F_aero_VSP]
  "Aerodynamic Forces and Moments "/2 -> [M_aero_VSP]
  Aerodynamic Forces and Moments 1/2 -> [M_aero_AVL]
  [F_aero_AVL] -> Switch/3
  [F_aero_VSP] -> Switch/1
  Switch/1 -> F_aero/1
  Switch1/1 -> M_aero/1
  [M_aero_VSP] -> Switch1/1
  [M_aero_AVL] -> Switch1/3
  b7/1 -> Switch/2
  b8/1 -> Switch1/2
  Aileron_R (deg)/1 -> Product/2, Abs/1
  Aeroelasticity_AIL/1 -> Product/1
  Abs/1 -> Aeroelasticity_AIL/1
  Product/1 -> [Ail_R_deg]
  Product1/1 -> [Ail_L_deg]
  Abs1/1 -> Aeroelasticity_AIL1/1
  Aeroelasticity_AIL1/1 -> Product1/1
  Aileron_L (deg)/1 -> Product1/2, Abs1/1
  Elevator (deg)/1 -> Abs2/1, Product2/2
  Aeroelasticity_ELE/1 -> Product2/1
  Abs2/1 -> Aeroelasticity_ELE/1
  Product2/1 -> [Ele_deg]
  Abs3/1 -> Aeroelasticity_RUD/1
  Rudder (deg)/1 -> Abs3/1, Product3/2
  Product3/1 -> [Rud_deg]
  Aeroelasticity_RUD/1 -> Product3/1
  Aerodynamic Forces and Moments 1/1 -> [F_aero_AVL]
  [CY] -> Mux3/2
  Gain15/1 -> CDD/9(Rud_deg)
  Gain4/1 -> CMl/9(Rud_deg)
  Gain9/1 -> CMm/9(Rud_deg)
  Gain10/1 -> CSS/9(Rud_deg)
  Gain11/1 -> CLL/9(Rud_deg)
  Gain12/1 -> CMn/9(Rud_deg)
  [uvw_m_s] -> "Aerodynamic Forces and Moments "/5
  Stab_r/1 -> [rs_rad_s]
  Stab_p/1 -> [ps_rad_s]
  Stab_Rate_In/1 -> Stab_r/1, Stab_p/1
  Degrees to Radians/1 -> Stab_Rate_In/3
  Demux1/1 -> Stab_Rate_In/1, [p_rad_s]
  Demux1/3 -> Stab_Rate_In/2, [r_rad_s]

== system FW_SkySurfer_HIL/UAV/UAV/Environment ==
  note: for Software Development Verification, comment through the transfer function
      | since the FixedStepDiscrete solver should be used without continuous states
  WIND_IDX : Inport
  wind.Vel : Inport  Port=2
  wind.Psi : Inport  Port=3
  Gravity : Subsystem
  ISA Atmosphere Model : aerolibatmos2/ISA Atmosphere Model  useExtended=off  action=Warning  custom=off  viscosityOut=off  g=9.80665  gamma=1.4  R=287.0531  L=0.0065  h_trop=11000  h_strat=20000  rho0=1.225  P0=101325  T0=288.15  h0=0  S=110.4  Tref=273.15  muref=1.716e-5
  Wind : Subsystem
  F_gravity : Outport  Unit=lbf
  Out Bus Element : Outport  Port=2  PortName=WIND  Element=UVW
  Out Bus Element1 : Outport  Port=2  PortName=WIND  Element=PQR
  tag scope: P_isa=global, T_isa=global, a=global, rho=global
  wires:
  [H] -> ISA Atmosphere Model/1
  Gravity/1(Gravity) -> F_gravity/1
  WIND_IDX/1 -> Wind/1(WIND_IDX)
  wind.Vel/1 -> Wind/2(wind.Vel)
  wind.Psi/1 -> Wind/3(wind.Psi)
  ISA Atmosphere Model/4 -> [rho]
  [DCM] -> Gravity/1(DCM)
  Wind/1(wind.UVW) -> Out Bus Element/1
  Wind/2(wind.PQR) -> Out Bus Element1/1
  ISA Atmosphere Model/2 -> [a]
  ISA Atmosphere Model/3 -> [P_isa]
  ISA Atmosphere Model/1 -> [T_isa]

== system FW_SkySurfer_HIL/UAV/UAV/Ground Model ==
  note: Body is assumed to be a rigid point mass on ground for contact force calculations.
      |
      | Normal force is modelled as a spring mass damper.
      |
      | Friction is modelled using Soft Coulomb model.
  DCMbe : Inport
  Xe : Inport  Port=2
  Ve : Inport  Port=3
  Friction Force : Subsystem
  Matrix Multiply : Product  Multiplication=Matrix(*)
  Mux1 : Mux  Inputs=2
  Normal Force : Subsystem
  Selector : Selector  InputPortWidth=3  IndexOptions=Index vector (dialog)  Indices=[3]  OutputSizes=1  RuntimeRangeChecks=off
  Selector1 : Selector  InputPortWidth=3  IndexOptions=Index vector (dialog)  Indices=[3]  OutputSizes=1  RuntimeRangeChecks=off
  Selector2 : Selector  InputPortWidth=3  IndexOptions=Index vector (dialog)  Indices=[1,2]  OutputSizes=1  RuntimeRangeChecks=off
  Unary Minus1 : UnaryMinus
  Fb_contact : Outport
  wires:
  Xe/1 -> Selector/1
  Ve/1 -> Selector2/1, Selector1/1
  Selector1/1 -> Normal Force/1(Vz)
  Selector/1 -> Normal Force/2(Z)
  DCMbe/1 -> Matrix Multiply/1
  Matrix Multiply/1 -> Fb_contact/1
  Normal Force/1(Normal) -> Friction Force/2(Fn), Unary Minus1/1
  Mux1/1 -> Matrix Multiply/2
  Unary Minus1/1 -> Mux1/2
  Selector2/1 -> Friction Force/1(V)
  Friction Force/1(Friction) -> Mux1/1

== system FW_SkySurfer_HIL/UAV/UAV/Measurement ==
  note: for Flying Quality Analysis,
      | use Continuous Derivative to obtain s-domain transfer function
  note: for Software Development Verification, comment through the transfer function
      | since the FixedStepDiscrete solver should be used without continuous states
  note: for Software Development Verification,
      | terminate the output since wind module contains continuous states
  Bus Element In : Inport  PortName=WIND  Element=UVW
  Bus Element In1 : Inport  PortName=WIND  Element=PQR
  Bus Element In7 : Inport  Port=2  PortName=INI_COND  Element=Latitude0
  Bus Element In2 : Inport  Port=2  PortName=INI_COND  Element=Longitude0
  VE : Inport  Port=3
  XE : Inport  Port=4
  EA : Inport  Port=5
  DCM : Inport  Port=6
  VB : Inport  Port=7
  AR : Inport  Port=8
  AB : Inport  Port=9
  AA : Inport  Port=10
  Q0123 : Inport  Port=11
  Add1 : Sum  Inputs=-+
  Add4 : Sum
  Dot Product : DotProduct  OutDataTypeStr=Inherit: Inherit via internal rule
  Mach Number : aerolibasang/Mach Number
  Negate_D_to_Alt : Gain  Gain=-1
  Radians to Degrees4 : simulink_extras/Transformations/Radians to Degrees
  Radians to Degrees5 : simulink_extras/Transformations/Radians to Degrees
  Selector11 : Selector  InputPortWidth=3  IndexOptions=Index vector (dialog)  Indices=3  OutputSizes=1  RuntimeRangeChecks=off
  Sqrt : Sqrt
  Subsystem : Subsystem
  Term_AA : Terminator
  Term_AB : Terminator
  Term_Bus_Element_In2 : Terminator
  Term_Bus_Element_In7 : Terminator
  Term_EA : Terminator
  Term_Q0123 : Terminator
  tag scope: AoA=global, AoS=global, DCM=global, H=global, Mach=global, PQRc=global, U=global, UVWc=global, V=global
  wires:
  Bus Element In1/1 -> Add4/1
  Bus Element In/1 -> Add1/1
  DCM/1 -> [DCM]
  Add4/1 -> [PQRc]
  [a] -> Mach Number/2
  Bus Element In2/1 -> Term_Bus_Element_In2/1
  Bus Element In7/1 -> Term_Bus_Element_In7/1
  Selector11/1 -> Negate_D_to_Alt/1
  Dot Product/1 -> Sqrt/1
  VE/1 -> Dot Product/2, Dot Product/1
  Add1/1 -> Subsystem/1(Vb), Mach Number/1, [UVWc]
  AR/1 -> Add4/2
  VB/1 -> Add1/2
  Subsystem/3(V) -> [V]
  Subsystem/2(Beta) -> Radians to Degrees5/1
  Subsystem/1(Alpha) -> Radians to Degrees4/1
  Mach Number/1 -> [Mach]
  Radians to Degrees4/1 -> [AoA]
  Radians to Degrees5/1 -> [AoS]
  Negate_D_to_Alt/1 -> [H]
  Sqrt/1 -> [U]
  XE/1 -> Selector11/1
  EA/1 -> Term_EA/1
  AB/1 -> Term_AB/1
  AA/1 -> Term_AA/1
  Q0123/1 -> Term_Q0123/1

== system FW_SkySurfer_HIL/UAV/UAV/Propulsion ==
  Throttle (0-1) : Inport
  Constant{,4..6} (4 alike) : Constant  Value=0
  Constant1 : Constant  Value=del_z
  Gain : Gain  Gain=-1
  Gain1 : Gain  Gain=g
  Mux1 : Mux  Inputs=3
  Mux4 : Mux  Inputs=3
  Product : Product
  kgf : Gain  Gain=2.45
  F_thr : Outport  Unit=lbf
  M_thr : Outport  Port=2
  wires:
  Constant4/1 -> Mux4/1
  Mux4/1 -> M_thr/1
  Constant5/1 -> Mux1/2
  Constant/1 -> Mux4/3
  Constant6/1 -> Mux1/3
  Mux1/1 -> F_thr/1
  Throttle (0-1)/1 -> kgf/1
  Constant1/1 -> Product/2
  Product/1 -> Gain/1
  Gain/1 -> Mux4/2
  kgf/1 -> Gain1/1
  Gain1/1 -> Mux1/1, Product/1

== system FW_SkySurfer_HIL/UAV/UAV/Subsystem ==
  Bus Element In7 : Inport  PortName=INI_COND  Element=U0
  Bus Element In2 : Inport  PortName=INI_COND  Element=Inertia0
  Bus Element In3 : Inport  PortName=INI_COND  Element=Theta0
  Bus Element In1 : Inport  PortName=INI_COND  Element=Mass0
  Bus Element In8 : Inport  PortName=INI_COND  Element=Psi0
  Bus Element In4 : Inport  PortName=INI_COND  Element=Phi0
  Bus Element In5 : Inport  PortName=INI_COND  Element=V0
  Bus Element In6 : Inport  PortName=INI_COND  Element=W0
  Bus Element In10 : Inport  PortName=INI_COND  Element=Alt0
  Constant1 : Constant  Value=0
  Constant2 : Constant  Value=zeros(3)
  Degrees to Radians6 : simulink_extras/Transformations/Degrees to Radians
  Gain : Gain  Gain=-1
  Mux1 : Mux  Inputs=3
  Mux2 : Mux  Inputs=3
  Mux3 : Mux  Inputs=3
  rho_sealevel (slug/ft^3)2 : Constant  Value=0  OutDataTypeStr=Inherit: Inherit via back propagation
  m_dot : Outport
  mass : Outport  Port=2
  I_dot : Outport  Port=3
  I : Outport  Port=4
  VB0 : Outport  Port=5
  EA0 : Outport  Port=6
  XE0 : Outport  Port=7
  tag scope: mass=global
  wires:
  Degrees to Radians6/1 -> EA0/1
  Constant1/1 -> m_dot/1
  Constant2/1 -> I_dot/1
  Bus Element In2/1 -> I/1
  Bus Element In4/1 -> Mux1/1
  Bus Element In3/1 -> Mux1/2
  Bus Element In8/1 -> Mux1/3
  Mux1/1 -> Degrees to Radians6/1
  Bus Element In5/1 -> Mux3/2
  Bus Element In6/1 -> Mux3/3
  Mux2/1 -> XE0/1
  Bus Element In10/1 -> Gain/1
  Gain/1 -> Mux2/3
  rho_sealevel (slug/ft^3)2/1 -> Mux2/2, Mux2/1
  Bus Element In7/1 -> Mux3/1
  Bus Element In1/1 -> [mass], mass/1
  Mux3/1 -> VB0/1

== system FW_SkySurfer_HIL/UAV/UAV/6DoF/Subsystem ==
  p q r : Inport
  eul_0 : Inport  Port=2
  Q0123 : Integrator  InitialConditionSource=external
  Quaternions to Direction Cosine Matrix : sharedtransform/Quaternions to  Direction Cosine Matrix  aMode=aMode
  Quaternions to Rotation Angles : sharedtransform/Quaternions to Rotation Angles  rotationOrder=ZYX  aMode=aMode
  Rotation Angles to Quaternions : sharedtransform/Rotation Angles to Quaternions  rotationOrder=ZYX  aMode=aMode
  Selector : Selector  InputPortWidth=3  IndexOptions=Index vector (dialog)  Indices=[3 2 1]  OutputSizes=1  RuntimeRangeChecks=off
  Selector1 : Selector  InputPortWidth=3  IndexOptions=Index vector (dialog)  Indices=[3 2 1]  OutputSizes=1  RuntimeRangeChecks=off
  qdot : shared6dofsys/qdot  aMode=aMode
  DCM : Outport  VectorParamsAs1DForOutWhenUnconnected=off
  Euler : Outport  Port=2  VectorParamsAs1DForOutWhenUnconnected=off
  Q : Outport  Port=3  VectorParamsAs1DForOutWhenUnconnected=off
  wires:
  Quaternions to Rotation Angles/1 -> Selector/1
  Selector/1 -> Euler/1
  p q r/1 -> qdot/1
  Selector1/1 -> Rotation Angles to Quaternions/1
  Quaternions to Direction Cosine Matrix/1 -> DCM/1
  eul_0/1 -> Selector1/1
  qdot/1 -> Q0123/1
  Rotation Angles to Quaternions/1 -> Q0123/2
  Q0123/1 -> Q/1, qdot/2, Quaternions to Rotation Angles/1, Quaternions to Direction Cosine Matrix/1

== system FW_SkySurfer_HIL/UAV/UAV/6DoF/Subsystem1 ==
  Vre : Inport  OutDataTypeStr=double
  forces : Inport  Port=2
  "mass " : Inport  Port=3
  mdot : Inport  Port=4
  I : Inport  Port=5
  I_dot : Inport  Port=6
  Ground : Ground
  Mass input/output momentum : shared6dofsys/Mass & Inertia (custom)/Mass input//output  momentum  SystemSampleTime=-1  VariantActivationTime=update diagram  EmptyChoice=off  PassThrough=off  PassThroughVariantControl=(default)  EmptyChoiceVariantControl=(default)  AllowFlexibleInterface=on  Latency=0  AutoFrameSizeCalculation=off
  Matrix Concatenation : Concatenate  Mode=Multidimensional array
  Reshape : Reshape
  Sum1 : Sum  Commented=on  Inputs=|++  SaturateOnIntegerOverflow=on
  Terminator : Terminator  Commented=on
  Terminator1 : Terminator
  "forces " : Outport  PortDimensions=3  VectorParamsAs1DForOutWhenUnconnected=off
  mass : Outport  Port=2  VectorParamsAs1DForOutWhenUnconnected=off
  "I, I_dot " : Outport  Port=3  VectorParamsAs1DForOutWhenUnconnected=off
  Out1 : Outport  Port=4  OutDataTypeStr=double  VectorParamsAs1DForOutWhenUnconnected=off
  wires:
  Ground/1 -> Out1/1
  I/1 -> Matrix Concatenation/1
  Matrix Concatenation/1 -> "I, I_dot "/1
  "mass "/1 -> mass/1
  Mass input/output momentum/1 -> Reshape/1
  I_dot/1 -> Matrix Concatenation/2
  mdot/1 -> Mass input/output momentum/2
  forces/1 -> "forces "/1, Sum1/1
  Vre/1 -> Mass input/output momentum/1
  Sum1/1 -> Terminator/1
  Reshape/1 -> Terminator1/1

== system FW_SkySurfer_HIL/UAV/UAV/6DoF/Subsystem2 ==
  p q r : Inport
  "I, I_dot" : Inport  Port=2
  Moments : Inport  Port=3
  3x3 Cross Product : sharedutil/3x3 Cross Product  aMode=aMode
  I x w : shared6dofsys/Calculate omega_dot/I x w  SystemSampleTime=-1  VariantActivationTime=update diagram  EmptyChoice=off  PassThrough=off  PassThroughVariantControl=(default)  EmptyChoiceVariantControl=(default)  AllowFlexibleInterface=on  Latency=0  AutoFrameSizeCalculation=off
  I x w1 : shared6dofsys/Calculate omega_dot/I x w1  SystemSampleTime=-1  VariantActivationTime=update diagram  EmptyChoice=off  PassThrough=off  PassThroughVariantControl=(default)  EmptyChoiceVariantControl=(default)  AllowFlexibleInterface=on  Latency=0  AutoFrameSizeCalculation=off
  Product2 : Product  Inputs=*/  Multiplication=Matrix(*)  SaturateOnIntegerOverflow=on  OutDataTypeStr=Inherit: Same as first input
  Reshape : Reshape
  Reshape1 : Reshape  OutputDimensionality=Row vector (2-D)
  Selector : Selector  NumberOfDimensions=2  InputPortWidth=2  IndexOptions=Index vector (dialog),Select all  Indices=1:3,-1  OutputSizes=1  RuntimeRangeChecks=off
  Selector1 : Selector  NumberOfDimensions=2  InputPortWidth=2  IndexOptions=Index vector (dialog),Select all  Indices=4:6,-1  OutputSizes=1  RuntimeRangeChecks=off
  Selector2 : Selector  NumberOfDimensions=2  InputPortWidth=2  IndexOptions=Index vector (dialog),Select all  Indices=1:3,-1  OutputSizes=1  RuntimeRangeChecks=off
  Sum2 : Sum  Inputs=+--  SaturateOnIntegerOverflow=on
  pdot qdot rdot : Outport  VectorParamsAs1DForOutWhenUnconnected=off
  wires:
  p q r/1 -> I x w1/2, 3x3 Cross Product/1, I x w/1
  3x3 Cross Product/1 -> Sum2/3
  Sum2/1 -> Reshape1/1
  Reshape1/1 -> Product2/1
  Selector1/1 -> I x w1/1
  Reshape/1 -> pdot qdot rdot/1
  "I, I_dot"/1 -> Selector1/1, Selector2/1, Selector/1
  Selector/1 -> I x w/2
  Product2/1 -> Reshape/1
  Moments/1 -> Sum2/1
  I x w1/1 -> Sum2/2
  Selector2/1 -> Product2/2
  I x w/1 -> 3x3 Cross Product/2

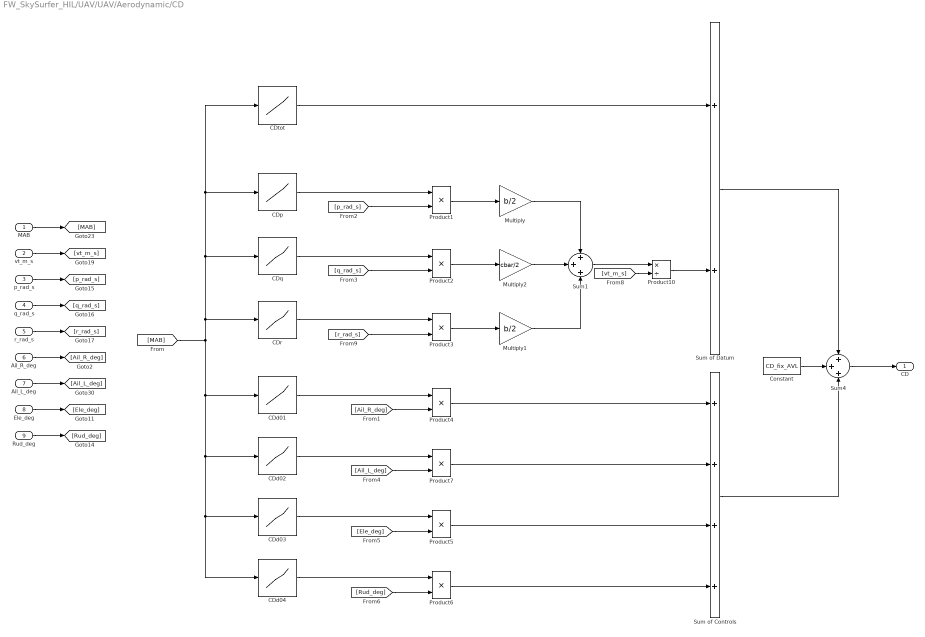
== system FW_SkySurfer_HIL/UAV/UAV/Aerodynamic/CD ==
  MAB : Inport
  vt_m_s : Inport  Port=2
  p_rad_s : Inport  Port=3
  q_rad_s : Inport  Port=4
  r_rad_s : Inport  Port=5
  Ail_R_deg : Inport  Port=6
  Ail_L_deg : Inport  Port=7
  Ele_deg : Inport  Port=8
  Rud_deg : Inport  Port=9
  CDd01 : Lookup_n-D  NumberOfTableDimensions=3  BreakpointsForDimension1=mach_avl  BreakpointsForDimension2=alpha_avl  BreakpointsForDimension3=beta_avl  UseOneInputPortForAllInputData=on  Table=CDd01  InternalRulePriority=Speed  RndMeth=Simplest
  CDd02 : Lookup_n-D  NumberOfTableDimensions=3  BreakpointsForDimension1=mach_avl  BreakpointsForDimension2=alpha_avl  BreakpointsForDimension3=beta_avl  UseOneInputPortForAllInputData=on  Table=CDd02  InternalRulePriority=Speed  RndMeth=Simplest
  CDd03 : Lookup_n-D  NumberOfTableDimensions=3  BreakpointsForDimension1=mach_avl  BreakpointsForDimension2=alpha_avl  BreakpointsForDimension3=beta_avl  UseOneInputPortForAllInputData=on  Table=CDd03  InternalRulePriority=Speed  RndMeth=Simplest
  CDd04 : Lookup_n-D  NumberOfTableDimensions=3  BreakpointsForDimension1=mach_avl  BreakpointsForDimension2=alpha_avl  BreakpointsForDimension3=beta_avl  UseOneInputPortForAllInputData=on  Table=CDd04  InternalRulePriority=Speed  RndMeth=Simplest
  CDp : Lookup_n-D  NumberOfTableDimensions=3  BreakpointsForDimension1=mach_avl  BreakpointsForDimension2=alpha_avl  BreakpointsForDimension3=beta_avl  UseOneInputPortForAllInputData=on  Table=CDp  ExtrapMethod=Clip  InternalRulePriority=Speed  RndMeth=Simplest
  CDq : Lookup_n-D  NumberOfTableDimensions=3  BreakpointsForDimension1=mach_avl  BreakpointsForDimension2=alpha_avl  BreakpointsForDimension3=beta_avl  UseOneInputPortForAllInputData=on  Table=CDq  InternalRulePriority=Speed  RndMeth=Simplest
  CDr : Lookup_n-D  NumberOfTableDimensions=3  BreakpointsForDimension1=mach_avl  BreakpointsForDimension2=alpha_avl  BreakpointsForDimension3=beta_avl  UseOneInputPortForAllInputData=on  Table=CDr  InternalRulePriority=Speed  RndMeth=Simplest
  CDtot : Lookup_n-D  NumberOfTableDimensions=3  BreakpointsForDimension1=mach_avl  BreakpointsForDimension2=alpha_avl  BreakpointsForDimension3=beta_avl  UseOneInputPortForAllInputData=on  Table=CDtot  ExtrapMethod=Clip  InternalRulePriority=Speed  RndMeth=Simplest
  Constant : Constant  Value=CD_fix_AVL
  Multiply : Gain  Gain=b/2
  Multiply1 : Gain  Gain=b/2
  Multiply2 : Gain  Gain=cbar/2
  Product{1..7} (7 alike) : Product
  Product10 : Product  Inputs=*/  InputSameDT=on  SaturateOnIntegerOverflow=on  OutDataTypeStr=Inherit: Same as first input
  Sum of Controls : Sum  Inputs=++++
  Sum of Datum : Sum
  Sum1 : Sum  Inputs=+++  InputSameDT=on  SaturateOnIntegerOverflow=on  OutDataTypeStr=Inherit: Same as first input
  Sum4 : Sum  Inputs=+++  InputSameDT=on  SaturateOnIntegerOverflow=on  OutDataTypeStr=Inherit: Same as first input
  CD : Outport
  wires:
  q_rad_s/1 -> [q_rad_s]
  Ail_R_deg/1 -> [Ail_R_deg]
  Ele_deg/1 -> [Ele_deg]
  MAB/1 -> [MAB]
  Ail_L_deg/1 -> [Ail_L_deg]
  p_rad_s/1 -> [p_rad_s]
  Rud_deg/1 -> [Rud_deg]
  r_rad_s/1 -> [r_rad_s]
  vt_m_s/1 -> [vt_m_s]
  Sum of Datum/1 -> Sum4/1
  Product4/1 -> Sum of Controls/1
  Product5/1 -> Sum of Controls/3
  CDq/1 -> Product2/1
  [q_rad_s] -> Product2/2
  CDd03/1 -> Product5/1
  [r_rad_s] -> Product3/2
  Product3/1 -> Multiply1/1
  CDp/1 -> Product1/1
  Product7/1 -> Sum of Controls/2
  CDr/1 -> Product3/1
  Product10/1 -> Sum of Datum/2
  Sum1/1 -> Product10/1
  CDd04/1 -> Product6/1
  CDtot/1 -> Sum of Datum/1
  [vt_m_s] -> Product10/2
  Multiply1/1 -> Sum1/3
  Product2/1 -> Multiply2/1
  CDd01/1 -> Product4/1
  Product6/1 -> Sum of Controls/4
  Multiply/1 -> Sum1/1
  Multiply2/1 -> Sum1/2
  Product1/1 -> Multiply/1
  [p_rad_s] -> Product1/2
  Sum4/1 -> CD/1
  Sum of Controls/1 -> Sum4/3
  [MAB] -> CDr/1, CDq/1, CDp/1, CDtot/1, CDd01/1, CDd02/1, CDd04/1, CDd03/1
  CDd02/1 -> Product7/1
  Constant/1 -> Sum4/2
  [Ail_L_deg] -> Product7/2
  [Rud_deg] -> Product6/2
  [Ele_deg] -> Product5/2
  [Ail_R_deg] -> Product4/2
